simulink model "CombinedExperiment"  (R2020a)
settings: Solver=FixedStepAuto  StartTime=0.0  StopTime=tsim  FixedStep=baseRate  RelTol=1e-3  EnableMultiTasking=on
values from neighbouring files (symbols this model uses):
  baseRate = 0.1    [Run_Initializer.m]
  drop_states_BLACK = [1.36947387695313,1.22175756835938,-0.0161599479615688]    [Run_Initializer.m]
  drop_states_BLUE = [ xLength/2+0.9; yLength/2+0.5; 0]    [Run_Initializer.m]
  drop_states_RED = [ xLength/2+1.1; yLength/2; pi]    [Run_Initializer.m]
  F_thrusters_BLACK = 0.25.*ones(8,1)    [Run_Initializer.m]
  F_thrusters_BLUE = 0.25.*ones(8,1)    [Run_Initializer.m]
  F_thrusters_RED = 0.25.*ones(8,1)    [Run_Initializer.m]
  home_states_BLACK = [ xLength/2; yLength/2; 0]    [Run_Initializer.m]
  home_states_BLUE = [ xLength/2-0.9; yLength/2+0.5; 0]    [Run_Initializer.m]
  home_states_RED = [ xLength/2+1.1; yLength/2; pi]    [Run_Initializer.m]
  init_states_BLACK = [ xLength/2; yLength/2; 0]    [Run_Initializer.m]
  init_states_BLUE = [ xLength/2+0.9; yLength/2+0.5; 0]    [Run_Initializer.m]
  init_states_RED = [ xLength/2+1.1; yLength/2; pi]    [Run_Initializer.m]
  Kd_tb = 0.4    [Run_Initializer.m]
  Kd_tblue = 0.4    [Run_Initializer.m]
  Kd_tr = 0.4    [Run_Initializer.m]
  Kd_xb = 5    [Run_Initializer.m]
  Kd_xblue = 5    [Run_Initializer.m]
  Kd_xr = 5    [Run_Initializer.m]
  Kd_yb = 5    [Run_Initializer.m]
  Kd_yblue = 5    [Run_Initializer.m]
  Kd_yr = 5    [Run_Initializer.m]
  Kp_tb = 0.1    [Run_Initializer.m]
  Kp_tblue = 0.1    [Run_Initializer.m]
  Kp_tr = 0.1    [Run_Initializer.m]
  Kp_xb = 2    [Run_Initializer.m]
  Kp_xblue = 2    [Run_Initializer.m]
  Kp_xr = 2    [Run_Initializer.m]
  Kp_yb = 2    [Run_Initializer.m]
  Kp_yblue = 2    [Run_Initializer.m]
  Kp_yr = 2    [Run_Initializer.m]
  noise_variance_BLACK = 0    [Run_Initializer.m]
  noise_variance_BLUE = 0    [Run_Initializer.m]
  noise_variance_RED = 0    [Run_Initializer.m]
  Phase0_End = Phase0_Duration    (= 10)    [Run_Initializer.m]
  Phase1_End = Phase0_Duration + Phase1_Duration    (= 15)    [Run_Initializer.m]
  Phase2_End = Phase0_Duration + Phase1_Duration +                                   Phase2_Duration    (= 40)    [Run_Initializer.m]
  Phase3_End = Phase0_Duration + Phase1_Duration +                                   Phase2_Duration + Phase3_Duration    (= 117)    [Run_Initializer.m]
  Phase3_SubPhase1_End = Phase2_End + Phase3_SubPhase1_Duration    (= 41)    [Run_Initializer.m]
  Phase3_SubPhase2_End = Phase2_End + Phase3_SubPhase1_Duration +                                   Phase3_SubPhase2_Duration    (= 42)    [Run_Initializer.m]
  Phase3_SubPhase3_End = Phase2_End + Phase3_SubPhase1_Duration +                                   Phase3_SubPhase2_Duration +                                  Phase3_SubPhase3_Duration    (= 72)    [Run_Initializer.m]
  Phase3_SubPhase4_End = Phase2_End + Phase3_SubPhase1_Duration +                                   Phase3_SubPhase2_Duration +                                  Phase3_SubPhase3_Duration +                                  Phase3_SubPhase4_Duration    [Run_Initializer.m]
  Phase4_End = Phase0_Duration + Phase1_Duration +                                   Phase2_Duration + Phase3_Duration +                                   Phase4_Duration    (= 137)    [Run_Initializer.m]
  Phase5_End = Phase0_Duration + Phase1_Duration +                                   Phase2_Duration + Phase3_Duration +                                   Phase4_Duration + Phase5_Duration    (= 142)    [Run_Initializer.m]
  serverRate = 0.2    [Run_Initializer.m]
  thruster_dist2CG_BLACK = [83.42;-52.58;55.94;-60.05;54.08;-53.92;77.06;-55.94]    [Run_Initializer.m]
  thruster_dist2CG_BLUE = [83.42;-52.58;55.94;-60.05;54.08;-53.92;77.06;-55.94]    [Run_Initializer.m]
  thruster_dist2CG_RED = [49.92;-78.08;70.46;-63.54;81.08;-50.42;57.44;-75.96]    [Run_Initializer.m]
  xLength = 3.51155    [Run_Initializer.m]
  yLength = 2.41935    [Run_Initializer.m]
undefined symbols (not defined in the file or in its folder): DiscIntNeverNeededParam, platformSelection, simMode, WhoAmI
libraries: dspstat3 x18, raspberrypiBasiclib x10, dspsigops x9, embdlinuxlib x8, simulink x8, MainLibrary x5, mspfiltlib x3, dsparch4 x3, dspswit3 x2, sensehatlib x1
(part 1 of 9)
settings Model: ExtModeTrigDuration=2  Creator=AlexC  LastModifiedBy=SPOT
settings SolverCC: PositivePriorityOrder=on
settings DataIOCC: ReturnWorkspaceOutputs=off
settings OptimizationCC: ZeroExternalMemoryAtStartup=off  ZeroInternalMemoryAtStartup=off  MaxStackSize=64
settings DebuggingCC: MultiTaskDSMMsg=none  ParameterTunabilityLossMsg=error  ArithmeticOperatorsInVariantConditions=warning
settings HardwareCC: ProdBitPerPointer=32  ProdBitPerSizeT=32  ProdBitPerPtrDiffT=32  ProdLargestAtomicInteger=Long  ProdLargestAtomicFloat=Double  ProdWordSize=32  ProdLongLongMode=on  ProdHWDeviceType=ARM Compatible->ARM Cortex
settings SFSimCC: CustomCodeUndefinedFunction=UseInterfaceOnly
settings RTWCC: SystemTargetFile=ert.tlc  HardwareBoard=Raspberry Pi  TemplateMakefile=ert_default_tmf  Toolchain=GNU GCC Raspberry Pi  BuildConfiguration=Faster Runs  TargetLang=C++
settings CodeAppCC: ForceParamTrailComments=on  OperatorAnnotations=on  StateflowObjectComments=on  MATLABSourceComments=on
settings ERTTargetCC: CodeReplacementLibrary=GCC ARM Cortex-A8  ERTCustomFileBanners=off  MatFileLogging=on  SupportContinuousTime=on  SupportNonInlinedSFcns=on  RemoveResetFunc=off  SupportVariableSizeSignals=on

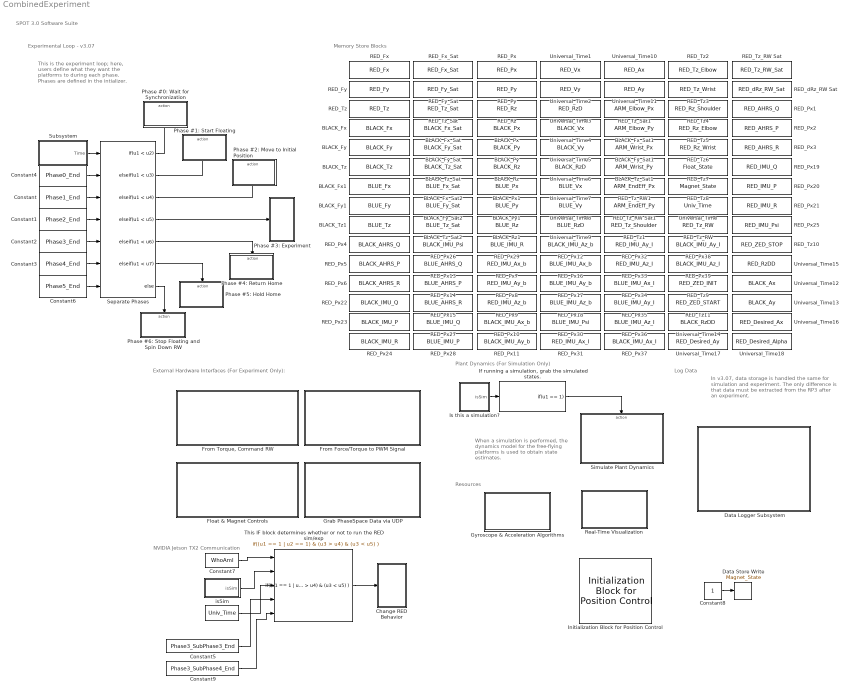
== system CombinedExperiment ==
  note: In v3.07, data storage is handled the same for simulation and experiment. The only difference is that data must be extracted from the RP3 after an experiment.
  note: Plant Dynamics (For Simulation Only)
  note: Log Data
  note: This is the experiment loop; here, users define what they want the platforms to during each phase. Phases are defined in the intializer.
  note: Memory Store Blocks
  note: Resources
  note: Experimental Loop - v3.07
  note: External Hardware Interfaces (For Experiment Only):
  note: SPOT 3.0
      | Software Suite
  note: When a simulation is performed, the dynamics model for the free-flying platforms is used to obtain state estimates.
  note: NVIDIA Jetson TX2 Communication
  " " : DataStoreRead  DataStoreName=Univ_Time
  BLACK_Fx : DataStoreMemory  DataStoreName=BLACK_Fx  ReadBeforeWriteMsg=warning  WriteAfterWriteMsg=warning  WriteAfterReadMsg=warning  ShowAdditionalParam=off
  BLACK_Fx1 : DataStoreMemory  DataStoreName=BLUE_Fx  ReadBeforeWriteMsg=warning  WriteAfterWriteMsg=warning  WriteAfterReadMsg=warning  ShowAdditionalParam=off
  BLACK_Fx_Sat : DataStoreMemory  DataStoreName=BLACK_Fx_Sat  ReadBeforeWriteMsg=warning  WriteAfterWriteMsg=warning  WriteAfterReadMsg=warning  ShowAdditionalParam=off
  BLACK_Fx_Sat1 : DataStoreMemory  DataStoreName=ARM_Elbow_Py  ReadBeforeWriteMsg=warning  WriteAfterWriteMsg=warning  WriteAfterReadMsg=warning  ShowAdditionalParam=off
  BLACK_Fx_Sat2 : DataStoreMemory  DataStoreName=BLUE_Fx_Sat  ReadBeforeWriteMsg=warning  WriteAfterWriteMsg=warning  WriteAfterReadMsg=warning  ShowAdditionalParam=off
  BLACK_Fy : DataStoreMemory  DataStoreName=BLACK_Fy  ReadBeforeWriteMsg=warning  WriteAfterWriteMsg=warning  WriteAfterReadMsg=warning  ShowAdditionalParam=off
  BLACK_Fy1 : DataStoreMemory  DataStoreName=BLUE_Fy  ReadBeforeWriteMsg=warning  WriteAfterWriteMsg=warning  WriteAfterReadMsg=warning  ShowAdditionalParam=off
  BLACK_Fy_Sat : DataStoreMemory  DataStoreName=BLACK_Fy_Sat  ReadBeforeWriteMsg=warning  WriteAfterWriteMsg=warning  WriteAfterReadMsg=warning  ShowAdditionalParam=off
  BLACK_Fy_Sat1 : DataStoreMemory  DataStoreName=ARM_Wrist_Px  ReadBeforeWriteMsg=warning  WriteAfterWriteMsg=warning  WriteAfterReadMsg=warning  ShowAdditionalParam=off
  BLACK_Fy_Sat2 : DataStoreMemory  DataStoreName=BLUE_Fy_Sat  ReadBeforeWriteMsg=warning  WriteAfterWriteMsg=warning  WriteAfterReadMsg=warning  ShowAdditionalParam=off
  BLACK_Px : DataStoreMemory  DataStoreName=BLACK_Px  ReadBeforeWriteMsg=warning  WriteAfterWriteMsg=warning  WriteAfterReadMsg=warning  ShowAdditionalParam=off
  BLACK_Px1 : DataStoreMemory  DataStoreName=BLUE_Px  ReadBeforeWriteMsg=warning  WriteAfterWriteMsg=warning  WriteAfterReadMsg=warning  ShowAdditionalParam=off
  BLACK_Py : DataStoreMemory  DataStoreName=BLACK_Py  ReadBeforeWriteMsg=warning  WriteAfterWriteMsg=warning  WriteAfterReadMsg=warning  ShowAdditionalParam=off
  BLACK_Py1 : DataStoreMemory  DataStoreName=BLUE_Py  ReadBeforeWriteMsg=warning  WriteAfterWriteMsg=warning  WriteAfterReadMsg=warning  ShowAdditionalParam=off
  BLACK_Rz : DataStoreMemory  DataStoreName=BLACK_Rz  ReadBeforeWriteMsg=warning  WriteAfterWriteMsg=warning  WriteAfterReadMsg=warning  ShowAdditionalParam=off
  BLACK_Rz1 : DataStoreMemory  DataStoreName=BLUE_Rz  ReadBeforeWriteMsg=warning  WriteAfterWriteMsg=warning  WriteAfterReadMsg=warning  ShowAdditionalParam=off
  BLACK_Tz : DataStoreMemory  DataStoreName=BLACK_Tz  ReadBeforeWriteMsg=warning  WriteAfterWriteMsg=warning  WriteAfterReadMsg=warning  ShowAdditionalParam=off
  BLACK_Tz1 : DataStoreMemory  DataStoreName=BLUE_Tz  ReadBeforeWriteMsg=warning  WriteAfterWriteMsg=warning  WriteAfterReadMsg=warning  ShowAdditionalParam=off
  BLACK_Tz_Sat : DataStoreMemory  DataStoreName=BLACK_Tz_Sat  ReadBeforeWriteMsg=warning  WriteAfterWriteMsg=warning  WriteAfterReadMsg=warning  ShowAdditionalParam=off
  BLACK_Tz_Sat1 : DataStoreMemory  DataStoreName=ARM_Wrist_Py  ReadBeforeWriteMsg=warning  WriteAfterWriteMsg=warning  WriteAfterReadMsg=warning  ShowAdditionalParam=off
  BLACK_Tz_Sat2 : DataStoreMemory  DataStoreName=BLUE_Tz_Sat  ReadBeforeWriteMsg=warning  WriteAfterWriteMsg=warning  WriteAfterReadMsg=warning  ShowAdditionalParam=off
  Change RED Behavior : Subsystem  TreatAsAtomicUnit=on
  Constant : Constant  Value=Phase1_End  SampleTime=-1
  Constant1 : Constant  Value=Phase2_End  SampleTime=-1
  Constant2 : Constant  Value=Phase3_End  SampleTime=-1
  Constant3 : Constant  Value=Phase4_End  SampleTime=-1
  Constant4 : Constant  Value=Phase0_End  SampleTime=-1
  Constant5 : Constant  Value=Phase3_SubPhase3_End
  Constant6 : Constant  Value=Phase5_End  SampleTime=-1
  Constant7 : Constant  Value=WhoAmI
  Constant8 : Constant
  Constant9 : Constant  Value=Phase3_SubPhase4_End
  Data Logger Subsystem : Subsystem
  Data Store Write : DataStoreWrite  DataStoreName=Magnet_State
  Float & Magnet Controls : Subsystem
  From Force/Torque to PWM Signal : Subsystem  SystemSampleTime=0.1
  "From Torque, Command RW" : Subsystem
  Grab PhaseSpace Data via UDP : Subsystem
  Gyroscope & Acceleration Algorithms : Subsystem
  "If running a simulation, grab the simulated states." : If  IfExpression=u1 == 1  ShowElse=off
  Initialization Block for Position Control : MainLibrary/Dynamixel Functions/Initialization Block for Position Control  P_GAIN=400  I_GAIN=0  D_GAIN=200  MAX_POSITION=4095  MIN_POSITION=0  VELOCITY_LIMIT=380
      settings: SourceProductName=SPOT Custom Library
  Is this a simulation? : Subsystem
  Phase #0: Wait for Synchronization : Subsystem  TreatAsAtomicUnit=on
  "Phase #1: Start Floating " : Subsystem  TreatAsAtomicUnit=on
  Phase #2: Move to Initial Position : Subsystem  TreatAsAtomicUnit=on
  Phase #3: Experiment : Subsystem  TreatAsAtomicUnit=on
  Phase #4: Return Home : Subsystem  TreatAsAtomicUnit=on
  Phase #5: Hold Home : Subsystem  TreatAsAtomicUnit=on
  Phase #6: Stop Floating and Spin Down RW : Subsystem  TreatAsAtomicUnit=on
  RED_Fx : DataStoreMemory  DataStoreName=RED_Fx  ReadBeforeWriteMsg=warning  WriteAfterWriteMsg=warning  WriteAfterReadMsg=warning  ShowAdditionalParam=off
  RED_Fx_Sat : DataStoreMemory  DataStoreName=RED_Fx_Sat  ReadBeforeWriteMsg=warning  WriteAfterWriteMsg=warning  WriteAfterReadMsg=warning  ShowAdditionalParam=off
  RED_Fy : DataStoreMemory  DataStoreName=RED_Fy  ReadBeforeWriteMsg=warning  WriteAfterWriteMsg=warning  WriteAfterReadMsg=warning  ShowAdditionalParam=off
  RED_Fy_Sat : DataStoreMemory  DataStoreName=RED_Fy_Sat  ReadBeforeWriteMsg=warning  WriteAfterWriteMsg=warning  WriteAfterReadMsg=warning  ShowAdditionalParam=off
  RED_Px : DataStoreMemory  DataStoreName=RED_Px  ReadBeforeWriteMsg=warning  WriteAfterWriteMsg=warning  WriteAfterReadMsg=warning  ShowAdditionalParam=off
  RED_Px1 : DataStoreMemory  DataStoreName=RED_AHRS_Q  ReadBeforeWriteMsg=warning  WriteAfterWriteMsg=warning  WriteAfterReadMsg=warning  ShowAdditionalParam=off
  RED_Px10 : DataStoreMemory  DataStoreName=BLACK_IMU_Ax_b  ReadBeforeWriteMsg=warning  WriteAfterWriteMsg=warning  WriteAfterReadMsg=warning  ShowAdditionalParam=off
  RED_Px11 : DataStoreMemory  DataStoreName=BLACK_IMU_Ay_b  ReadBeforeWriteMsg=warning  WriteAfterWriteMsg=warning  WriteAfterReadMsg=warning  ShowAdditionalParam=off
  RED_Px12 : DataStoreMemory  DataStoreName=BLACK_IMU_Az_b  ReadBeforeWriteMsg=warning  WriteAfterWriteMsg=warning  WriteAfterReadMsg=warning  ShowAdditionalParam=off
  RED_Px13 : DataStoreMemory  DataStoreName=BLUE_AHRS_Q  ReadBeforeWriteMsg=warning  WriteAfterWriteMsg=warning  WriteAfterReadMsg=warning  ShowAdditionalParam=off
  RED_Px14 : DataStoreMemory  DataStoreName=BLUE_AHRS_P  ReadBeforeWriteMsg=warning  WriteAfterWriteMsg=warning  WriteAfterReadMsg=warning  ShowAdditionalParam=off
  RED_Px15 : DataStoreMemory  DataStoreName=BLUE_AHRS_R  ReadBeforeWriteMsg=warning  WriteAfterWriteMsg=warning  WriteAfterReadMsg=warning  ShowAdditionalParam=off
  RED_Px16 : DataStoreMemory  DataStoreName=BLUE_IMU_Ax_b  ReadBeforeWriteMsg=warning  WriteAfterWriteMsg=warning  WriteAfterReadMsg=warning  ShowAdditionalParam=off
  RED_Px17 : DataStoreMemory  DataStoreName=BLUE_IMU_Ay_b  ReadBeforeWriteMsg=warning  WriteAfterWriteMsg=warning  WriteAfterReadMsg=warning  ShowAdditionalParam=off
  RED_Px18 : DataStoreMemory  DataStoreName=BLUE_IMU_Az_b  ReadBeforeWriteMsg=warning  WriteAfterWriteMsg=warning  WriteAfterReadMsg=warning  ShowAdditionalParam=off
  RED_Px19 : DataStoreMemory  DataStoreName=RED_IMU_Q  ReadBeforeWriteMsg=warning  WriteAfterWriteMsg=warning  WriteAfterReadMsg=warning  ShowAdditionalParam=off
  RED_Px2 : DataStoreMemory  DataStoreName=RED_AHRS_P  ReadBeforeWriteMsg=warning  WriteAfterWriteMsg=warning  WriteAfterReadMsg=warning  ShowAdditionalParam=off
  RED_Px20 : DataStoreMemory  DataStoreName=RED_IMU_P  ReadBeforeWriteMsg=warning  WriteAfterWriteMsg=warning  WriteAfterReadMsg=warning  ShowAdditionalParam=off
  RED_Px21 : DataStoreMemory  DataStoreName=RED_IMU_R  ReadBeforeWriteMsg=warning  WriteAfterWriteMsg=warning  WriteAfterReadMsg=warning  ShowAdditionalParam=off
  RED_Px22 : DataStoreMemory  DataStoreName=BLACK_IMU_Q  ReadBeforeWriteMsg=warning  WriteAfterWriteMsg=warning  WriteAfterReadMsg=warning  ShowAdditionalParam=off
  RED_Px23 : DataStoreMemory  DataStoreName=BLACK_IMU_P  ReadBeforeWriteMsg=warning  WriteAfterWriteMsg=warning  WriteAfterReadMsg=warning  ShowAdditionalParam=off
  RED_Px24 : DataStoreMemory  DataStoreName=BLACK_IMU_R  ReadBeforeWriteMsg=warning  WriteAfterWriteMsg=warning  WriteAfterReadMsg=warning  ShowAdditionalParam=off
  RED_Px25 : DataStoreMemory  DataStoreName=RED_IMU_Psi  ReadBeforeWriteMsg=warning  WriteAfterWriteMsg=warning  WriteAfterReadMsg=warning  ShowAdditionalParam=off
  RED_Px26 : DataStoreMemory  DataStoreName=BLACK_IMU_Psi  ReadBeforeWriteMsg=warning  WriteAfterWriteMsg=warning  WriteAfterReadMsg=warning  ShowAdditionalParam=off
  RED_Px27 : DataStoreMemory  DataStoreName=BLUE_IMU_Q  ReadBeforeWriteMsg=warning  WriteAfterWriteMsg=warning  WriteAfterReadMsg=warning  ShowAdditionalParam=off
  RED_Px28 : DataStoreMemory  DataStoreName=BLUE_IMU_P  ReadBeforeWriteMsg=warning  WriteAfterWriteMsg=warning  WriteAfterReadMsg=warning  ShowAdditionalParam=off
  RED_Px29 : DataStoreMemory  DataStoreName=BLUE_IMU_R  ReadBeforeWriteMsg=warning  WriteAfterWriteMsg=warning  WriteAfterReadMsg=warning  ShowAdditionalParam=off
  RED_Px3 : DataStoreMemory  DataStoreName=RED_AHRS_R  ReadBeforeWriteMsg=warning  WriteAfterWriteMsg=warning  WriteAfterReadMsg=warning  ShowAdditionalParam=off
  RED_Px30 : DataStoreMemory  DataStoreName=BLUE_IMU_Psi  ReadBeforeWriteMsg=warning  WriteAfterWriteMsg=warning  WriteAfterReadMsg=warning  ShowAdditionalParam=off
  RED_Px31 : DataStoreMemory  DataStoreName=RED_IMU_Ax_I  ReadBeforeWriteMsg=warning  WriteAfterWriteMsg=warning  WriteAfterReadMsg=warning  ShowAdditionalParam=off
  RED_Px32 : DataStoreMemory  DataStoreName=RED_IMU_Ay_I  ReadBeforeWriteMsg=warning  WriteAfterWriteMsg=warning  WriteAfterReadMsg=warning  ShowAdditionalParam=off
  RED_Px33 : DataStoreMemory  DataStoreName=RED_IMU_Az_I  ReadBeforeWriteMsg=warning  WriteAfterWriteMsg=warning  WriteAfterReadMsg=warning  ShowAdditionalParam=off
  RED_Px34 : DataStoreMemory  DataStoreName=BLUE_IMU_Ax_I  ReadBeforeWriteMsg=warning  WriteAfterWriteMsg=warning  WriteAfterReadMsg=warning  ShowAdditionalParam=off
  RED_Px35 : DataStoreMemory  DataStoreName=BLUE_IMU_Ay_I  ReadBeforeWriteMsg=warning  WriteAfterWriteMsg=warning  WriteAfterReadMsg=warning  ShowAdditionalParam=off
  RED_Px36 : DataStoreMemory  DataStoreName=BLUE_IMU_Az_I  ReadBeforeWriteMsg=warning  WriteAfterWriteMsg=warning  WriteAfterReadMsg=warning  ShowAdditionalParam=off
  RED_Px37 : DataStoreMemory  DataStoreName=BLACK_IMU_Ax_I  ReadBeforeWriteMsg=warning  WriteAfterWriteMsg=warning  WriteAfterReadMsg=warning  ShowAdditionalParam=off
  RED_Px38 : DataStoreMemory  DataStoreName=BLACK_IMU_Ay_I  ReadBeforeWriteMsg=warning  WriteAfterWriteMsg=warning  WriteAfterReadMsg=warning  ShowAdditionalParam=off
  RED_Px39 : DataStoreMemory  DataStoreName=BLACK_IMU_Az_I  ReadBeforeWriteMsg=warning  WriteAfterWriteMsg=warning  WriteAfterReadMsg=warning  ShowAdditionalParam=off
  RED_Px4 : DataStoreMemory  DataStoreName=BLACK_AHRS_Q  ReadBeforeWriteMsg=warning  WriteAfterWriteMsg=warning  WriteAfterReadMsg=warning  ShowAdditionalParam=off
  RED_Px5 : DataStoreMemory  DataStoreName=BLACK_AHRS_P  ReadBeforeWriteMsg=warning  WriteAfterWriteMsg=warning  WriteAfterReadMsg=warning  ShowAdditionalParam=off
  RED_Px6 : DataStoreMemory  DataStoreName=BLACK_AHRS_R  ReadBeforeWriteMsg=warning  WriteAfterWriteMsg=warning  WriteAfterReadMsg=warning  ShowAdditionalParam=off
  RED_Px7 : DataStoreMemory  DataStoreName=RED_IMU_Ax_b  ReadBeforeWriteMsg=warning  WriteAfterWriteMsg=warning  WriteAfterReadMsg=warning  ShowAdditionalParam=off
  RED_Px8 : DataStoreMemory  DataStoreName=RED_IMU_Ay_b  ReadBeforeWriteMsg=warning  WriteAfterWriteMsg=warning  WriteAfterReadMsg=warning  ShowAdditionalParam=off
  RED_Px9 : DataStoreMemory  DataStoreName=RED_IMU_Az_b  ReadBeforeWriteMsg=warning  WriteAfterWriteMsg=warning  WriteAfterReadMsg=warning  ShowAdditionalParam=off
  RED_Py : DataStoreMemory  DataStoreName=RED_Py  ReadBeforeWriteMsg=warning  WriteAfterWriteMsg=warning  WriteAfterReadMsg=warning  ShowAdditionalParam=off
  RED_Rz : DataStoreMemory  DataStoreName=RED_Rz  ReadBeforeWriteMsg=warning  WriteAfterWriteMsg=warning  WriteAfterReadMsg=warning  ShowAdditionalParam=off
  RED_Tz : DataStoreMemory  DataStoreName=RED_Tz  ReadBeforeWriteMsg=warning  WriteAfterWriteMsg=warning  WriteAfterReadMsg=warning  ShowAdditionalParam=off
  RED_Tz1 : DataStoreMemory  DataStoreName=RED_Tz_Shoulder  ReadBeforeWriteMsg=warning  WriteAfterWriteMsg=warning  WriteAfterReadMsg=warning  ShowAdditionalParam=off
  RED_Tz10 : DataStoreMemory  DataStoreName=RED_ZED_STOP  ReadBeforeWriteMsg=warning  WriteAfterWriteMsg=warning  WriteAfterReadMsg=warning  ShowAdditionalParam=off
  RED_Tz11 : DataStoreMemory  DataStoreName=RED_ZED_START  ReadBeforeWriteMsg=warning  WriteAfterWriteMsg=warning  WriteAfterReadMsg=warning  ShowAdditionalParam=off
  RED_Tz2 : DataStoreMemory  DataStoreName=RED_Tz_Elbow  ReadBeforeWriteMsg=warning  WriteAfterWriteMsg=warning  WriteAfterReadMsg=warning  ShowAdditionalParam=off
  RED_Tz3 : DataStoreMemory  DataStoreName=RED_Tz_Wrist  ReadBeforeWriteMsg=warning  WriteAfterWriteMsg=warning  WriteAfterReadMsg=warning  ShowAdditionalParam=off
  RED_Tz4 : DataStoreMemory  DataStoreName=RED_Rz_Shoulder  ReadBeforeWriteMsg=warning  WriteAfterWriteMsg=warning  WriteAfterReadMsg=warning  ShowAdditionalParam=off
  RED_Tz5 : DataStoreMemory  DataStoreName=RED_Rz_Elbow  ReadBeforeWriteMsg=warning  WriteAfterWriteMsg=warning  WriteAfterReadMsg=warning  ShowAdditionalParam=off
  RED_Tz6 : DataStoreMemory  DataStoreName=RED_Rz_Wrist  ReadBeforeWriteMsg=warning  WriteAfterWriteMsg=warning  WriteAfterReadMsg=warning  ShowAdditionalParam=off
  RED_Tz7 : DataStoreMemory  DataStoreName=Float_State  ReadBeforeWriteMsg=warning  WriteAfterWriteMsg=warning  WriteAfterReadMsg=warning  ShowAdditionalParam=off
  RED_Tz8 : DataStoreMemory  DataStoreName=Magnet_State  ReadBeforeWriteMsg=warning  WriteAfterWriteMsg=warning  WriteAfterReadMsg=warning  ShowAdditionalParam=off
  RED_Tz9 : DataStoreMemory  DataStoreName=RED_ZED_INIT  ReadBeforeWriteMsg=warning  WriteAfterWriteMsg=warning  WriteAfterReadMsg=warning  ShowAdditionalParam=off
  RED_Tz_RW : DataStoreMemory  DataStoreName=RED_Tz_RW  ReadBeforeWriteMsg=warning  WriteAfterWriteMsg=warning  WriteAfterReadMsg=warning  ShowAdditionalParam=off
  RED_Tz_RW Sat : DataStoreMemory  DataStoreName=RED_Tz_RW_Sat  ReadBeforeWriteMsg=warning  WriteAfterWriteMsg=warning  WriteAfterReadMsg=warning  ShowAdditionalParam=off
  RED_Tz_RW Sat1 : DataStoreMemory  DataStoreName=ARM_EndEff_Py  ReadBeforeWriteMsg=warning  WriteAfterWriteMsg=warning  WriteAfterReadMsg=warning  ShowAdditionalParam=off
  RED_Tz_RW1 : DataStoreMemory  DataStoreName=ARM_EndEff_Px  ReadBeforeWriteMsg=warning  WriteAfterWriteMsg=warning  WriteAfterReadMsg=warning  ShowAdditionalParam=off
  RED_Tz_Sat : DataStoreMemory  DataStoreName=RED_Tz_Sat  ReadBeforeWriteMsg=warning  WriteAfterWriteMsg=warning  WriteAfterReadMsg=warning  ShowAdditionalParam=off
  RED_Tz_Sat1 : DataStoreMemory  DataStoreName=ARM_Elbow_Px  ReadBeforeWriteMsg=warning  WriteAfterWriteMsg=warning  WriteAfterReadMsg=warning  ShowAdditionalParam=off
  RED_dRz_RW Sat : DataStoreMemory  DataStoreName=RED_dRz_RW_Sat  ReadBeforeWriteMsg=warning  WriteAfterWriteMsg=warning  WriteAfterReadMsg=warning  ShowAdditionalParam=off
  Real-Time Visualization : Subsystem
  Separate Phases : If  NumInputs=7  IfExpression=u1 < u2  ElseIfExpressions=u1 < u3, u1 < u4, u1 < u5, u1 < u6, u1 < u7
  Simulate Plant Dynamics : Subsystem  TreatAsAtomicUnit=on
  Subsystem : Subsystem
  "This IF block determines whether or not to run the RED sim/exp " : If  NumInputs=5  IfExpression=(u1 == 1 | u2 == 1) & (u3 > u4) & (u3 < u5)  ShowElse=off
  Universal_Time : DataStoreMemory  DataStoreName=Univ_Time  ReadBeforeWriteMsg=warning  WriteAfterWriteMsg=warning  WriteAfterReadMsg=warning  ShowAdditionalParam=off
  Universal_Time1 : DataStoreMemory  DataStoreName=RED_Vx  ReadBeforeWriteMsg=warning  WriteAfterWriteMsg=warning  WriteAfterReadMsg=warning  ShowAdditionalParam=off
  Universal_Time10 : DataStoreMemory  DataStoreName=RED_Ax  ReadBeforeWriteMsg=warning  WriteAfterWriteMsg=warning  WriteAfterReadMsg=warning  ShowAdditionalParam=off
  Universal_Time11 : DataStoreMemory  DataStoreName=RED_Ay  ReadBeforeWriteMsg=warning  WriteAfterWriteMsg=warning  WriteAfterReadMsg=warning  ShowAdditionalParam=off
  Universal_Time12 : DataStoreMemory  DataStoreName=BLACK_Ax  ReadBeforeWriteMsg=warning  WriteAfterWriteMsg=warning  WriteAfterReadMsg=warning  ShowAdditionalParam=off
  Universal_Time13 : DataStoreMemory  DataStoreName=BLACK_Ay  ReadBeforeWriteMsg=warning  WriteAfterWriteMsg=warning  WriteAfterReadMsg=warning  ShowAdditionalParam=off
  Universal_Time14 : DataStoreMemory  DataStoreName=BLACK_RzDD  ReadBeforeWriteMsg=warning  WriteAfterWriteMsg=warning  WriteAfterReadMsg=warning  ShowAdditionalParam=off
  Universal_Time15 : DataStoreMemory  DataStoreName=RED_RzDD  ReadBeforeWriteMsg=warning  WriteAfterWriteMsg=warning  WriteAfterReadMsg=warning  ShowAdditionalParam=off
  Universal_Time16 : DataStoreMemory  DataStoreName=RED_Desired_Ax  ReadBeforeWriteMsg=warning  WriteAfterWriteMsg=warning  WriteAfterReadMsg=warning  ShowAdditionalParam=off
  Universal_Time17 : DataStoreMemory  DataStoreName=RED_Desired_Ay  ReadBeforeWriteMsg=warning  WriteAfterWriteMsg=warning  WriteAfterReadMsg=warning  ShowAdditionalParam=off
  Universal_Time18 : DataStoreMemory  DataStoreName=RED_Desired_Alpha  ReadBeforeWriteMsg=warning  WriteAfterWriteMsg=warning  WriteAfterReadMsg=warning  ShowAdditionalParam=off
  Universal_Time2 : DataStoreMemory  DataStoreName=RED_Vy  ReadBeforeWriteMsg=warning  WriteAfterWriteMsg=warning  WriteAfterReadMsg=warning  ShowAdditionalParam=off
  Universal_Time3 : DataStoreMemory  DataStoreName=RED_RzD  ReadBeforeWriteMsg=warning  WriteAfterWriteMsg=warning  WriteAfterReadMsg=warning  ShowAdditionalParam=off
  Universal_Time4 : DataStoreMemory  DataStoreName=BLACK_Vx  ReadBeforeWriteMsg=warning  WriteAfterWriteMsg=warning  WriteAfterReadMsg=warning  ShowAdditionalParam=off
  Universal_Time5 : DataStoreMemory  DataStoreName=BLACK_Vy  ReadBeforeWriteMsg=warning  WriteAfterWriteMsg=warning  WriteAfterReadMsg=warning  ShowAdditionalParam=off
  Universal_Time6 : DataStoreMemory  DataStoreName=BLACK_RzD  ReadBeforeWriteMsg=warning  WriteAfterWriteMsg=warning  WriteAfterReadMsg=warning  ShowAdditionalParam=off
  Universal_Time7 : DataStoreMemory  DataStoreName=BLUE_Vx  ReadBeforeWriteMsg=warning  WriteAfterWriteMsg=warning  WriteAfterReadMsg=warning  ShowAdditionalParam=off
  Universal_Time8 : DataStoreMemory  DataStoreName=BLUE_Vy  ReadBeforeWriteMsg=warning  WriteAfterWriteMsg=warning  WriteAfterReadMsg=warning  ShowAdditionalParam=off
  Universal_Time9 : DataStoreMemory  DataStoreName=BLUE_RzD  ReadBeforeWriteMsg=warning  WriteAfterWriteMsg=warning  WriteAfterReadMsg=warning  ShowAdditionalParam=off
  isSim : Subsystem
  wires:
  Constant4/1 -> Separate Phases/2
  Separate Phases/2 -> "Phase #1: Start Floating "/Action
  "If running a simulation, grab the simulated states."/1 -> Simulate Plant Dynamics/Action
  Constant/1 -> Separate Phases/3
  Constant1/1 -> Separate Phases/4
  Separate Phases/7 -> Phase #6: Stop Floating and Spin Down RW/Action
  Constant3/1 -> Separate Phases/6
  Separate Phases/3 -> Phase #2: Move to Initial Position/Action
  Separate Phases/1 -> Phase #0: Wait for Synchronization/Action
  Is this a simulation?/1(isSim) -> "If running a simulation, grab the simulated states."/1
  Constant2/1 -> Separate Phases/5
  Constant6/1 -> Separate Phases/7
  Separate Phases/6 -> Phase #5: Hold Home/Action
  Separate Phases/5 -> Phase #4: Return Home/Action
  Subsystem/1(Time) -> Separate Phases/1
  Separate Phases/4 -> Phase #3: Experiment/Action
  Constant5/1 -> "This IF block determines whether or not to run the RED sim/exp "/4
  " "/1 -> "This IF block determines whether or not to run the RED sim/exp "/3
  isSim/1(isSim) -> "This IF block determines whether or not to run the RED sim/exp "/2
  Constant7/1 -> "This IF block determines whether or not to run the RED sim/exp "/1
  "This IF block determines whether or not to run the RED sim/exp "/1 -> Change RED Behavior/Action
  Constant8/1 -> Data Store Write/1
  Constant9/1 -> "This IF block determines whether or not to run the RED sim/exp "/5

== system CombinedExperiment/Change RED Behavior ==
  Action Port : ActionPort  ActionPortLabel=if((u1 == 1 | u2 == 1) & (u3 > u4) & (u3 < u5) )
  " " : DataStoreRead  DataStoreName=Univ_Time
  Add : Sum  Inputs=+-
  Constant5 : Constant  Value=Phase3_SubPhase3_End
  Data Store Read : DataStoreRead  DataStoreName=RED_Px
  Data Store Read1 : DataStoreRead  DataStoreName=RED_Py
  Data Store Read10 : DataStoreRead  DataStoreName=BLACK_Vy
  Data Store Read11 : DataStoreRead  DataStoreName=BLACK_RzD
  Data Store Read2 : DataStoreRead  DataStoreName=RED_Rz
  Data Store Read3 : DataStoreRead  DataStoreName=BLACK_Px
  Data Store Read4 : DataStoreRead  DataStoreName=BLACK_Py
  Data Store Read5 : DataStoreRead  DataStoreName=BLACK_Rz
  Data Store Read6 : DataStoreRead  DataStoreName=RED_Vx
  Data Store Read7 : DataStoreRead  DataStoreName=RED_Vy
  Data Store Read8 : DataStoreRead  DataStoreName=RED_RzD
  Data Store Read9 : DataStoreRead  DataStoreName=BLACK_Vx
  Data Store Write3 : DataStoreWrite  DataStoreName=RED_Desired_Ax
  Data Store Write4 : DataStoreWrite  DataStoreName=RED_Desired_Ay
  Data Store Write5 : DataStoreWrite  DataStoreName=RED_Desired_Alpha
  MATLAB System : MATLABSystem  System=guidance_server
      mask Type: guidance_server
      mask Display: disp('guidance_server');
  wires:
  Data Store Read1/1 -> MATLAB System/3
  Data Store Read/1 -> MATLAB System/2
  Data Store Read2/1 -> MATLAB System/4
  Data Store Read3/1 -> MATLAB System/8
  Data Store Read4/1 -> MATLAB System/9
  Data Store Read5/1 -> MATLAB System/10
  MATLAB System/1 -> Data Store Write3/1
  MATLAB System/2 -> Data Store Write4/1
  MATLAB System/3 -> Data Store Write5/1
  Data Store Read6/1 -> MATLAB System/5
  Data Store Read7/1 -> MATLAB System/6
  Data Store Read8/1 -> MATLAB System/7
  Data Store Read9/1 -> MATLAB System/11
  Data Store Read10/1 -> MATLAB System/12
  Data Store Read11/1 -> MATLAB System/13
  " "/1 -> Add/1
  Add/1 -> MATLAB System/1
  Constant5/1 -> Add/2

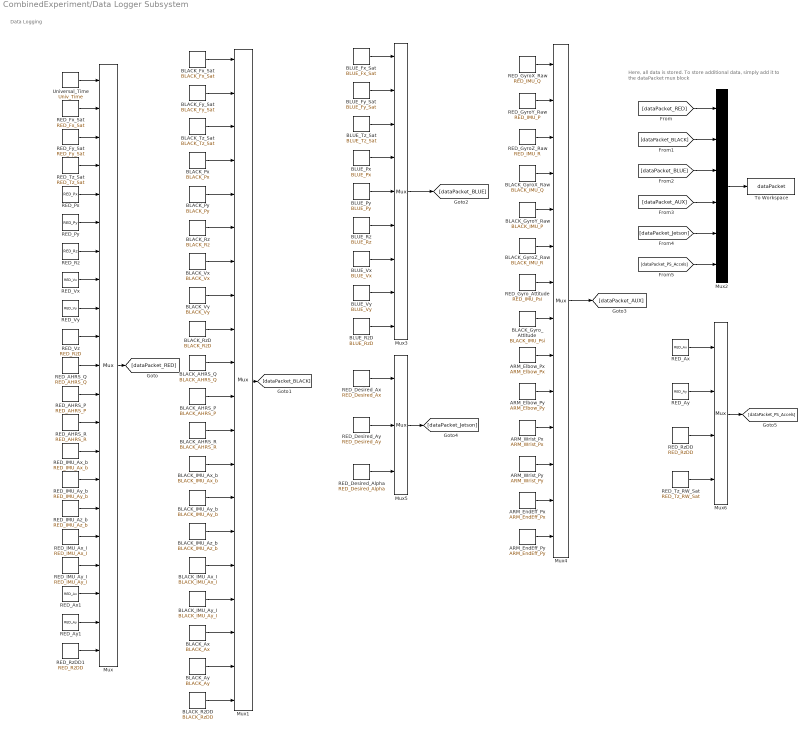
== system CombinedExperiment/Data Logger Subsystem ==
  note: Data Logging
  note: Here, all data is stored. To store additional data, simply add it to the dataPacket mux block
  ARM_Elbow_Px : DataStoreRead  DataStoreName=ARM_Elbow_Px
  ARM_Elbow_Py : DataStoreRead  DataStoreName=ARM_Elbow_Py
  ARM_EndEff_Px : DataStoreRead  DataStoreName=ARM_EndEff_Px
  ARM_EndEff_Py : DataStoreRead  DataStoreName=ARM_EndEff_Py
  ARM_Wrist_Px : DataStoreRead  DataStoreName=ARM_Wrist_Px
  ARM_Wrist_Py : DataStoreRead  DataStoreName=ARM_Wrist_Py
  BLACK_AHRS_P : DataStoreRead  DataStoreName=BLACK_AHRS_P
  BLACK_AHRS_Q : DataStoreRead  DataStoreName=BLACK_AHRS_Q
  BLACK_AHRS_R : DataStoreRead  DataStoreName=BLACK_AHRS_R
  BLACK_Ax : DataStoreRead  DataStoreName=BLACK_Ax
  BLACK_Ay : DataStoreRead  DataStoreName=BLACK_Ay
  BLACK_Fx_Sat : DataStoreRead  DataStoreName=BLACK_Fx_Sat
  BLACK_Fy_Sat : DataStoreRead  DataStoreName=BLACK_Fy_Sat
  BLACK_GyroX_Raw : DataStoreRead  DataStoreName=BLACK_IMU_Q
  BLACK_GyroY_Raw : DataStoreRead  DataStoreName=BLACK_IMU_P
  BLACK_GyroZ_Raw : DataStoreRead  DataStoreName=BLACK_IMU_R
  BLACK_Gyro_Attitude : DataStoreRead  DataStoreName=BLACK_IMU_Psi
  BLACK_IMU_Ax_I : DataStoreRead  DataStoreName=BLACK_IMU_Ax_I
  BLACK_IMU_Ax_b : DataStoreRead  DataStoreName=BLACK_IMU_Ax_b
  BLACK_IMU_Ay_I : DataStoreRead  DataStoreName=BLACK_IMU_Ay_I
  BLACK_IMU_Ay_b : DataStoreRead  DataStoreName=BLACK_IMU_Ay_b
  BLACK_IMU_Az_b : DataStoreRead  DataStoreName=BLACK_IMU_Az_b
  BLACK_Px : DataStoreRead  DataStoreName=BLACK_Px
  BLACK_Py : DataStoreRead  DataStoreName=BLACK_Py
  BLACK_Rz : DataStoreRead  DataStoreName=BLACK_Rz
  BLACK_RzD : DataStoreRead  DataStoreName=BLACK_RzD
  BLACK_RzDD : DataStoreRead  DataStoreName=BLACK_RzDD
  BLACK_Tz_Sat : DataStoreRead  DataStoreName=BLACK_Tz_Sat
  BLACK_Vx : DataStoreRead  DataStoreName=BLACK_Vx
  BLACK_Vy : DataStoreRead  DataStoreName=BLACK_Vy
  BLUE_Fx_Sat : DataStoreRead  DataStoreName=BLUE_Fx_Sat
  BLUE_Fy_Sat : DataStoreRead  DataStoreName=BLUE_Fy_Sat
  BLUE_Px : DataStoreRead  DataStoreName=BLUE_Px
  BLUE_Py : DataStoreRead  DataStoreName=BLUE_Py
  BLUE_Rz : DataStoreRead  DataStoreName=BLUE_Rz
  BLUE_RzD : DataStoreRead  DataStoreName=BLUE_RzD
  BLUE_Tz_Sat : DataStoreRead  DataStoreName=BLUE_Tz_Sat
  BLUE_Vx : DataStoreRead  DataStoreName=BLUE_Vx
  BLUE_Vy : DataStoreRead  DataStoreName=BLUE_Vy
  Mux : Mux  Inputs=21
  Mux1 : Mux  Inputs=20
  Mux2 : Mux  Inputs=6
  Mux3 : Mux  Inputs=9
  Mux4 : Mux  Inputs=14
  Mux5 : Mux  Inputs=3
  Mux6 : Mux
  RED_AHRS_P : DataStoreRead  DataStoreName=RED_AHRS_P
  RED_AHRS_Q : DataStoreRead  DataStoreName=RED_AHRS_Q
  RED_AHRS_R : DataStoreRead  DataStoreName=RED_AHRS_R
  RED_Ax : DataStoreRead  DataStoreName=RED_Ax
  RED_Ax1 : DataStoreRead  DataStoreName=RED_Ax
  RED_Ay : DataStoreRead  DataStoreName=RED_Ay
  RED_Ay1 : DataStoreRead  DataStoreName=RED_Ay
  RED_Desired_Alpha : DataStoreRead  DataStoreName=RED_Desired_Alpha
  RED_Desired_Ax : DataStoreRead  DataStoreName=RED_Desired_Ax
  RED_Desired_Ay : DataStoreRead  DataStoreName=RED_Desired_Ay
  RED_Fx_Sat : DataStoreRead  DataStoreName=RED_Fx_Sat
  RED_Fy_Sat : DataStoreRead  DataStoreName=RED_Fy_Sat
  RED_GyroX_Raw : DataStoreRead  DataStoreName=RED_IMU_Q
  RED_GyroY_Raw : DataStoreRead  DataStoreName=RED_IMU_P
  RED_GyroZ_Raw : DataStoreRead  DataStoreName=RED_IMU_R
  RED_Gyro_Attitude : DataStoreRead  DataStoreName=RED_IMU_Psi
  RED_IMU_Ax_I : DataStoreRead  DataStoreName=RED_IMU_Ax_I
  RED_IMU_Ax_b : DataStoreRead  DataStoreName=RED_IMU_Ax_b
  RED_IMU_Ay_I : DataStoreRead  DataStoreName=RED_IMU_Ay_I
  RED_IMU_Ay_b : DataStoreRead  DataStoreName=RED_IMU_Ay_b
  RED_IMU_Az_b : DataStoreRead  DataStoreName=RED_IMU_Az_b
  RED_Px : DataStoreRead  DataStoreName=RED_Px
  "RED_Py " : DataStoreRead  DataStoreName=RED_Py
  RED_Rz : DataStoreRead  DataStoreName=RED_Rz
  RED_RzDD : DataStoreRead  DataStoreName=RED_RzDD
  RED_RzDD1 : DataStoreRead  DataStoreName=RED_RzDD
  RED_Tz_RW_Sat : DataStoreRead  DataStoreName=RED_Tz_RW_Sat
  RED_Tz_Sat : DataStoreRead  DataStoreName=RED_Tz_Sat
  "RED_Vx " : DataStoreRead  DataStoreName=RED_Vx
  RED_Vy : DataStoreRead  DataStoreName=RED_Vy
  RED_Vz : DataStoreRead  DataStoreName=RED_RzD
  To Workspace : ToWorkspace  VariableName=dataPacket  SampleTime=-1
      settings: Save2DSignal=2-D array (concatenate along first dimension)
  Universal_Time : DataStoreRead  DataStoreName=Univ_Time
  wires:
  [dataPacket_BLACK] -> Mux2/2
  [dataPacket_RED] -> Mux2/1
  Mux2/1 -> To Workspace/1
  Mux3/1 -> [dataPacket_BLUE]
  BLUE_Tz_Sat/1 -> Mux3/3
  BLUE_RzD/1 -> Mux3/9
  BLUE_Fx_Sat/1 -> Mux3/1
  BLUE_Fy_Sat/1 -> Mux3/2
  BLUE_Px/1 -> Mux3/4
  BLUE_Vy/1 -> Mux3/8
  BLUE_Rz/1 -> Mux3/6
  BLUE_Py/1 -> Mux3/5
  BLUE_Vx/1 -> Mux3/7
  [dataPacket_BLUE] -> Mux2/3
  Mux4/1 -> [dataPacket_AUX]
  RED_GyroX_Raw/1 -> Mux4/1
  RED_GyroY_Raw/1 -> Mux4/2
  RED_GyroZ_Raw/1 -> Mux4/3
  [dataPacket_AUX] -> Mux2/4
  BLACK_GyroX_Raw/1 -> Mux4/4
  BLACK_GyroY_Raw/1 -> Mux4/5
  BLACK_GyroZ_Raw/1 -> Mux4/6
  RED_Gyro_Attitude/1 -> Mux4/7
  BLACK_Gyro_Attitude/1 -> Mux4/8
  ARM_Wrist_Py/1 -> Mux4/12
  ARM_EndEff_Px/1 -> Mux4/13
  ARM_EndEff_Py/1 -> Mux4/14
  ARM_Wrist_Px/1 -> Mux4/11
  ARM_Elbow_Py/1 -> Mux4/10
  ARM_Elbow_Px/1 -> Mux4/9
  RED_Desired_Ax/1 -> Mux5/1
  RED_Desired_Ay/1 -> Mux5/2
  RED_Desired_Alpha/1 -> Mux5/3
  Mux5/1 -> [dataPacket_Jetson]
  [dataPacket_Jetson] -> Mux2/5
  Mux6/1 -> [dataPacket_PS_Accels]
  RED_Ax/1 -> Mux6/1
  RED_Ay/1 -> Mux6/2
  RED_RzDD/1 -> Mux6/3
  [dataPacket_PS_Accels] -> Mux2/6
  RED_Tz_RW_Sat/1 -> Mux6/4
  BLACK_Ax/1 -> Mux1/18
  RED_Ay1/1 -> Mux/20
  BLACK_IMU_Ax_I/1 -> Mux1/16
  RED_RzDD1/1 -> Mux/21
  BLACK_AHRS_R/1 -> Mux1/12
  BLACK_Py/1 -> Mux1/5
  BLACK_AHRS_P/1 -> Mux1/11
  "RED_Vx "/1 -> Mux/8
  BLACK_AHRS_Q/1 -> Mux1/10
  BLACK_IMU_Ay_b/1 -> Mux1/14
  BLACK_RzDD/1 -> Mux1/20
  RED_IMU_Az_b/1 -> Mux/16
  RED_Ax1/1 -> Mux/19
  Mux/1 -> [dataPacket_RED]
  BLACK_Fx_Sat/1 -> Mux1/1
  RED_Fx_Sat/1 -> Mux/2
  BLACK_Fy_Sat/1 -> Mux1/2
  Mux1/1 -> [dataPacket_BLACK]
  BLACK_IMU_Ay_I/1 -> Mux1/17
  BLACK_Vx/1 -> Mux1/7
  RED_Rz/1 -> Mux/7
  BLACK_RzD/1 -> Mux1/9
  BLACK_Px/1 -> Mux1/4
  RED_IMU_Ay_I/1 -> Mux/18
  BLACK_IMU_Ax_b/1 -> Mux1/13
  BLACK_IMU_Az_b/1 -> Mux1/15
  "RED_Py "/1 -> Mux/6
  RED_Px/1 -> Mux/5
  BLACK_Tz_Sat/1 -> Mux1/3
  RED_Tz_Sat/1 -> Mux/4
  RED_AHRS_Q/1 -> Mux/11
  RED_Vz/1 -> Mux/10
  RED_IMU_Ay_b/1 -> Mux/15
  RED_IMU_Ax_I/1 -> Mux/17
  BLACK_Rz/1 -> Mux1/6
  RED_AHRS_R/1 -> Mux/13
  RED_Vy/1 -> Mux/9
  RED_Fy_Sat/1 -> Mux/3
  RED_AHRS_P/1 -> Mux/12
  Universal_Time/1 -> Mux/1
  RED_IMU_Ax_b/1 -> Mux/14
  BLACK_Ay/1 -> Mux1/19
  BLACK_Vy/1 -> Mux1/8

== system CombinedExperiment/Float & Magnet Controls ==
  note: In this subsection, the "if" statements are used to determine two things: 1) whether or not a simulation is begin performed,
      | then 2) if an experiment is being performed, then which platform is the diagram compiled on. The "IdentifyPlatform" variable
      | is obtained from a text file location on each platform; each text file contains a unique identifier for each platform.
  Change Behavior : Subsystem  TreatAsAtomicUnit=on
  Is this a simulation? : Subsystem
  This IF block determines whether or not to run the exp code : If  IfExpression=u1 == 0  ShowElse=off
  wires:
  Is this a simulation?/1(isSim) -> This IF block determines whether or not to run the exp code/1
  This IF block determines whether or not to run the exp code/1 -> Change Behavior/Action

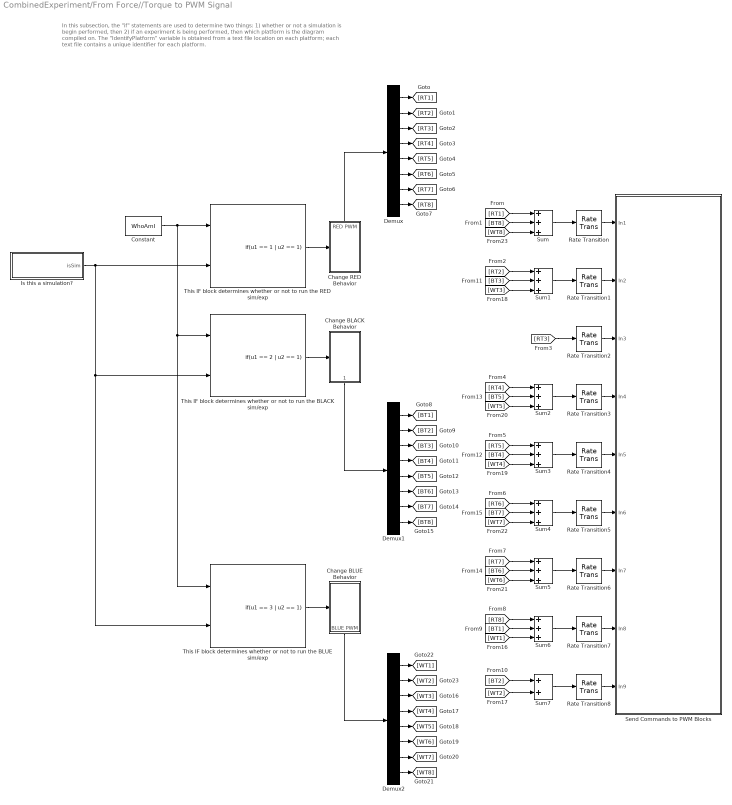
== system CombinedExperiment/From Force//Torque to PWM Signal ==
  note: In this subsection, the "if" statements are used to determine two things: 1) whether or not a simulation is begin performed,
      | then 2) if an experiment is being performed, then which platform is the diagram compiled on. The "IdentifyPlatform" variable
      | is obtained from a text file location on each platform; each text file contains a unique identifier for each platform.
  Change BLACK Behavior : Subsystem  TreatAsAtomicUnit=on
  Change BLUE Behavior : Subsystem  TreatAsAtomicUnit=on
  Change RED Behavior : Subsystem  TreatAsAtomicUnit=on
  Constant : Constant  Value=WhoAmI
  Demux : Demux  Outputs=8
  Demux1 : Demux  Outputs=8
  Demux2 : Demux  Outputs=8
  Is this a simulation? : Subsystem
  Rate Transition{,1..8} (9 alike) : RateTransition  OutPortSampleTime=0.1
  Send Commands to PWM Blocks : Subsystem  TreatAsAtomicUnit=on  SystemSampleTime=0.1
  Sum{,1..6} (7 alike) : Sum  Inputs=+++
  Sum7 : Sum
  This IF block determines whether or not to run the BLACK sim/exp : If  NumInputs=2  IfExpression=u1 == 2 | u2 == 1  ShowElse=off
  This IF block determines whether or not to run the BLUE sim/exp : If  NumInputs=2  IfExpression=u1 == 3 | u2 == 1  ShowElse=off
  "This IF block determines whether or not to run the RED sim/exp " : If  NumInputs=2  IfExpression=u1 == 1 | u2 == 1  ShowElse=off
  wires:
  Is this a simulation?/1(isSim) -> This IF block determines whether or not to run the BLACK sim/exp/2, This IF block determines whether or not to run the BLUE sim/exp/2, "This IF block determines whether or not to run the RED sim/exp "/2
  "This IF block determines whether or not to run the RED sim/exp "/1 -> Change RED Behavior/Action
  This IF block determines whether or not to run the BLACK sim/exp/1 -> Change BLACK Behavior/Action
  Change RED Behavior/1(RED PWM) -> Demux/1
  Demux/1 -> [RT1]
  Demux/2 -> [RT2]
  Demux/3 -> [RT3]
  Demux/4 -> [RT4]
  Demux/5 -> [RT5]
  Demux/6 -> [RT6]
  Demux/7 -> [RT7]
  Demux/8 -> [RT8]
  Demux1/5 -> [BT5]
  Demux1/4 -> [BT4]
  Demux1/1 -> [BT1]
  Demux1/8 -> [BT8]
  Demux1/2 -> [BT2]
  Demux1/7 -> [BT7]
  Demux1/6 -> [BT6]
  Demux1/3 -> [BT3]
  Change BLACK Behavior/1(BLACK PWM) -> Demux1/1
  [RT1] -> Sum/1
  [BT8] -> Sum/2
  [RT2] -> Sum1/1
  [RT4] -> Sum2/1
  [RT5] -> Sum3/1
  [RT6] -> Sum4/1
  [RT7] -> Sum5/1
  [RT8] -> Sum6/1
  [BT1] -> Sum6/2
  [BT3] -> Sum1/2
  [BT4] -> Sum3/2
  [BT5] -> Sum2/2
  [BT6] -> Sum5/2
  [BT7] -> Sum4/2
  Sum/1 -> Rate Transition/1
  Sum1/1 -> Rate Transition1/1
  [RT3] -> Rate Transition2/1
  Sum2/1 -> Rate Transition3/1
  Sum3/1 -> Rate Transition4/1
  Sum4/1 -> Rate Transition5/1
  Sum5/1 -> Rate Transition6/1
  Sum6/1 -> Rate Transition7/1
  Rate Transition/1 -> Send Commands to PWM Blocks/1(In1)
  Rate Transition1/1 -> Send Commands to PWM Blocks/2(In2)
  Rate Transition2/1 -> Send Commands to PWM Blocks/3(In3)
  Rate Transition3/1 -> Send Commands to PWM Blocks/4(In4)
  Rate Transition4/1 -> Send Commands to PWM Blocks/5(In5)
  Rate Transition5/1 -> Send Commands to PWM Blocks/6(In6)
  Rate Transition6/1 -> Send Commands to PWM Blocks/7(In7)
  Rate Transition7/1 -> Send Commands to PWM Blocks/8(In8)
  Rate Transition8/1 -> Send Commands to PWM Blocks/9(In9)
  Constant/1 -> This IF block determines whether or not to run the BLUE sim/exp/1, This IF block determines whether or not to run the BLACK sim/exp/1, "This IF block determines whether or not to run the RED sim/exp "/1
  This IF block determines whether or not to run the BLUE sim/exp/1 -> Change BLUE Behavior/Action
  Demux2/5 -> [WT5]
  Demux2/8 -> [WT8]
  Demux2/7 -> [WT7]
  Demux2/2 -> [WT2]
  Change BLUE Behavior/1(BLUE PWM) -> Demux2/1
  Demux2/1 -> [WT1]
  Demux2/4 -> [WT4]
  Demux2/3 -> [WT3]
  Demux2/6 -> [WT6]
  Sum7/1 -> Rate Transition8/1
  [BT2] -> Sum7/1
  [WT1] -> Sum6/3
  [WT2] -> Sum7/2
  [WT3] -> Sum1/3
  [WT4] -> Sum3/3
  [WT5] -> Sum2/3
  [WT6] -> Sum5/3
  [WT7] -> Sum4/3
  [WT8] -> Sum/3

== system CombinedExperiment/From Torque, Command RW ==
  note: In this subsection, the "if" statements are used to determine two things: 1) whether or not a simulation is begin performed,
      | then 2) if an experiment is being performed, then which platform is the diagram compiled on. The "IdentifyPlatform" variable
      | is obtained from a text file location on each platform; each text file contains a unique identifier for each platform.
  Change BLACK Behavior : Subsystem  TreatAsAtomicUnit=on
  Change BLUE Behavior : Subsystem  TreatAsAtomicUnit=on
  Change RED Behavior : Subsystem  TreatAsAtomicUnit=on
  Constant : Constant  Value=WhoAmI
  Is this a simulation? : Subsystem
  This IF block determines whether or not to run the BLACK sim/exp : If  NumInputs=2  IfExpression=u1 == 2 | u2 == 1  ShowElse=off
  This IF block determines whether or not to run the BLUE sim/exp : If  NumInputs=2  IfExpression=u1 == 3 | u2 == 1  ShowElse=off
  "This IF block determines whether or not to run the RED sim/exp " : If  NumInputs=2  IfExpression=u1 == 1 | u2 == 1  ShowElse=off
  wires:
  "This IF block determines whether or not to run the RED sim/exp "/1 -> Change RED Behavior/Action
  This IF block determines whether or not to run the BLACK sim/exp/1 -> Change BLACK Behavior/Action
  Is this a simulation?/1(isSim) -> This IF block determines whether or not to run the BLUE sim/exp/2, This IF block determines whether or not to run the BLACK sim/exp/2, "This IF block determines whether or not to run the RED sim/exp "/2
  This IF block determines whether or not to run the BLUE sim/exp/1 -> Change BLUE Behavior/Action
  Constant/1 -> This IF block determines whether or not to run the BLUE sim/exp/1, This IF block determines whether or not to run the BLACK sim/exp/1, "This IF block determines whether or not to run the RED sim/exp "/1

== system CombinedExperiment/Grab PhaseSpace Data via UDP ==
  "If performing an experiment, grab the PhaseSpace data. Otherwise, use a clock to set time in SIM." : If  IfExpression=u1 == 0  ElseIfExpressions=u1 == 1  ShowElse=off
  Initialize Universal Time (Simulation) : Subsystem  TreatAsAtomicUnit=on
  Is this a simulation?1 : Subsystem
  Use Hardware to Obtain States : Subsystem  TreatAsAtomicUnit=on
  wires:
  Is this a simulation?1/1(isSim) -> "If performing an experiment, grab the PhaseSpace data. Otherwise, use a clock to set time in SIM."/1
  "If performing an experiment, grab the PhaseSpace data. Otherwise, use a clock to set time in SIM."/2 -> Initialize Universal Time (Simulation)/Action
  "If performing an experiment, grab the PhaseSpace data. Otherwise, use a clock to set time in SIM."/1 -> Use Hardware to Obtain States/Action

== system CombinedExperiment/Gyroscope & Acceleration Algorithms ==
  Change BLACK Behavior : Subsystem  TreatAsAtomicUnit=on
  Change BLUE Behavior : Subsystem  TreatAsAtomicUnit=on
  Change RED Behavior : Subsystem  TreatAsAtomicUnit=on
  Constant1 : Constant  Value=WhoAmI
  Is this a simulation? : Subsystem
  LSM9DS1 IMU Sensor : sensehatlib/LSM9DS1 IMU Sensor  blockPlatform=Raspberry Pi  BoardProperty_sh=Pi 3 Model B  ActiveSensors_=Accelerometer, Gyroscope and Magnetometer  AccelerometerOutputDataRate=119 Hz  AccelerometerFullScaleRange=+/- 2g  AccelerometerBandwidth=50 Hz  GyroscopeOutputDataRate=119 Hz  GyroscopeFullScaleRange=245 dps  GyroscopeBandwidthMode=0  GyroscopeHighPassFilterEnabled=off  GyroscopeHighPassFilterMode=0  MagnetometerFullScaleRange=+/- 4 gauss  MagnetometerOutputDataRate=40 Hz  SampleTime=baseRate
      settings: SourceProductBaseCode=RASPPI
  Mux : Mux  Inputs=[3,3,3]
  This IF block determines whether or not to run the BLACK sim/exp : If  NumInputs=2  IfExpression=u1 == 2 & u2 == 0  ShowElse=off
  This IF block determines whether or not to run the BLUE sim/exp : If  NumInputs=2  IfExpression=u1 == 3 & u2 == 0  ShowElse=off
  "This IF block determines whether or not to run the RED sim/exp " : If  NumInputs=2  IfExpression=u1 == 1 & u2 ==0  ShowElse=off
  wires:
  "This IF block determines whether or not to run the RED sim/exp "/1 -> Change RED Behavior/Action
  This IF block determines whether or not to run the BLACK sim/exp/1 -> Change BLACK Behavior/Action
  Is this a simulation?/1(isSim) -> This IF block determines whether or not to run the BLACK sim/exp/2, This IF block determines whether or not to run the BLUE sim/exp/2, "This IF block determines whether or not to run the RED sim/exp "/2
  Constant1/1 -> This IF block determines whether or not to run the BLUE sim/exp/1, This IF block determines whether or not to run the BLACK sim/exp/1, "This IF block determines whether or not to run the RED sim/exp "/1
  This IF block determines whether or not to run the BLUE sim/exp/1 -> Change BLUE Behavior/Action
  LSM9DS1 IMU Sensor/1 -> Mux/1
  LSM9DS1 IMU Sensor/2 -> Mux/2
  LSM9DS1 IMU Sensor/3 -> Mux/3
  Mux/1 -> Change BLACK Behavior/1(IMU IN), Change RED Behavior/1(IMU IN), Change BLUE Behavior/1(IMU IN)

== system CombinedExperiment/Is this a simulation? ==
  Constant : Constant  Value=simMode  SampleTime=-1
  isSim : Outport  VectorParamsAs1DForOutWhenUnconnected=off
  wires:
  Constant/1 -> isSim/1

== system CombinedExperiment/Phase #0: Wait for Synchronization ==
  note: In this subsection, the "if" statements are used to determine two things: 1) whether or not a simulation is begin performed,
      | then 2) if an experiment is being performed, then which platform is the diagram compiled on. The "IdentifyPlatform" variable
      | is obtained from a text file location on each platform; each text file contains a unique identifier for each platform.
  Action Port : ActionPort  ActionPortLabel=if(u1 < u2)
  Change BLACK Behavior : Subsystem  TreatAsAtomicUnit=on
  Change BLUE Behavior : Subsystem  TreatAsAtomicUnit=on
  Change RED Behavior : Subsystem  TreatAsAtomicUnit=on
  Constant : Constant  Value=WhoAmI
  Is this a simulation? : Subsystem
  This IF block determines whether or not to run the BLACK sim/exp : If  NumInputs=2  IfExpression=u1 == 2 | u2 == 1  ShowElse=off
  This IF block determines whether or not to run the BLUE sim/exp : If  NumInputs=2  IfExpression=u1 == 3 | u2 == 1  ShowElse=off
  "This IF block determines whether or not to run the RED sim/exp " : If  NumInputs=2  IfExpression=u1 == 1 | u2 == 1  ShowElse=off
  wires:
  Is this a simulation?/1(isSim) -> This IF block determines whether or not to run the BLACK sim/exp/2, This IF block determines whether or not to run the BLUE sim/exp/2, "This IF block determines whether or not to run the RED sim/exp "/2
  "This IF block determines whether or not to run the RED sim/exp "/1 -> Change RED Behavior/Action
  This IF block determines whether or not to run the BLACK sim/exp/1 -> Change BLACK Behavior/Action
  Constant/1 -> This IF block determines whether or not to run the BLUE sim/exp/1, This IF block determines whether or not to run the BLACK sim/exp/1, "This IF block determines whether or not to run the RED sim/exp "/1
  This IF block determines whether or not to run the BLUE sim/exp/1 -> Change BLUE Behavior/Action

== system CombinedExperiment/Phase #1: Start Floating  ==
  note: In this subsection, the "if" statements are used to determine two things: 1) whether or not a simulation is begin performed,
      | then 2) if an experiment is being performed, then which platform is the diagram compiled on. The "IdentifyPlatform" variable
      | is obtained from a text file location on each platform; each text file contains a unique identifier for each platform.
  Action Port : ActionPort  ActionPortLabel=elseif(u1 < u3)
  Change BLACK Behavior : Subsystem  TreatAsAtomicUnit=on
  Change BLUE Behavior : Subsystem  TreatAsAtomicUnit=on
  Change RED Behavior : Subsystem  TreatAsAtomicUnit=on
  Constant : Constant  Value=WhoAmI
  Is this a simulation? : Subsystem
  This IF block determines whether or not to run the BLACK sim/exp : If  NumInputs=2  IfExpression=u1 == 2 | u2 == 1  ShowElse=off
  This IF block determines whether or not to run the BLUE sim/exp : If  NumInputs=2  IfExpression=u1 == 3 | u2 == 1  ShowElse=off
  "This IF block determines whether or not to run the RED sim/exp " : If  NumInputs=2  IfExpression=u1 == 1 | u2 == 1  ShowElse=off
  wires:
  "This IF block determines whether or not to run the RED sim/exp "/1 -> Change RED Behavior/Action
  This IF block determines whether or not to run the BLACK sim/exp/1 -> Change BLACK Behavior/Action
  Is this a simulation?/1(isSim) -> This IF block determines whether or not to run the BLUE sim/exp/2, This IF block determines whether or not to run the BLACK sim/exp/2, "This IF block determines whether or not to run the RED sim/exp "/2
  This IF block determines whether or not to run the BLUE sim/exp/1 -> Change BLUE Behavior/Action
  Constant/1 -> This IF block determines whether or not to run the BLUE sim/exp/1, This IF block determines whether or not to run the BLACK sim/exp/1, "This IF block determines whether or not to run the RED sim/exp "/1
